simulink model "DataCenterCooling"  (R2026a)
settings: Solver=VariableStepAuto  StopTime=432000  AbsTol=1e-3
PreLoadFcn:
  | load DataCenterCoolingHeatLoad.mat
  | load DataCenterCoolingEnviornment.mat
  | 
  | % Chiller Setpoint
  | T_chiller = 18; % degC
  | 
  | % Pipes
  | server_pipe_D = 0.02; % m
  | server_pipe_L = 12; % m
  | server_pipe_thickness = 0.002; % m
  | server_num_pipes = 800;
  | 
  | % Material properties
  | rho_pipe = 7800; % kg/m^3
  | cp_pipe = 500; % J/(kg*K)
  | 
  | % Total connecting port areas
  | port_area = 0.2; % m^2
  | 
  | % Cooling tower
  | T_reservoir = 23; % degC
  | fan_area = 15; % m^2
  | tower_height = 3; % m
  | tower_area = 15; % m^2
libraries: fl_lib x38, nesl_utility x24, SimscapeFluids_lib x14, simulink_extras x2, slpidlib x2
(part 1 of 2)
CloseFcn:
  | try,close(h1_DataCenterCooling),end
  | clear h1_DataCenterCooling
  | try,close(h2_DataCenterCooling),end
  | clear h2_DataCenterCooling
  | try,close(h3_DataCenterCooling),end
  | clear h3_DataCenterCooling
  | 
  | clear tout simlog_DataCenterCooling
  | clear heat_load environment
  | clear T_chiller server_pipe_D server_pipe_L server_pipe_thickness server_num_pipes
  | clear rho_pipe cp_pipe port_area T_reservoir fan_area tower_height tower_area
Description:
  | Data Center Cooling
settings Model: Creator=The MathWorks, Inc.
settings SolverCC: MaxConsecutiveMinStep=500
settings DataIOCC: ReturnWorkspaceOutputs=on  SignalLogging=on  SaveTime=on  SaveOutput=on
settings DebuggingCC: SymbolicDimsDataTypeCodeGenerationDiagnostic=none
settings SimscapeCC: SimscapeNominalValues="[{\"value\":\"1\",\"unit\":\"A\"},{\"value\":\"1\",\"unit\":\"bar\"},{\"value\":\"1\",\"unit\":\"cm^2\"},{\"value\":\"1\",\"unit\":\"cm^3/s\"},{\"value\":\"1\",\"unit\":\"kJ/kg\"},{\"value\":\"1\",\"unit\":\"kW\"},{\"value\":\"1\",\"unit\":\"l\"},{\"value\":\"1\",\"unit\":\"N\"},{\"value\":\"1\",\"unit\":\"N*m\"},{\"value\":\"1\",\"unit\":\"V\"}]"  SimscapeLogSimulationStatistics=on  SimscapeLogName=simlog_DataCenterCooling  SimscapeLogDataHistory=50000.0

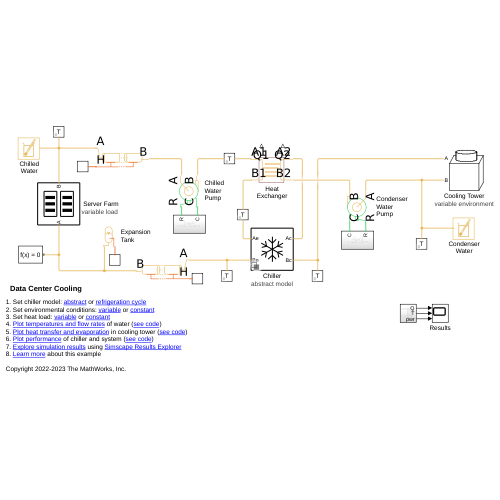
[thumbnail: Simulink's stored preview of the top-level diagram]
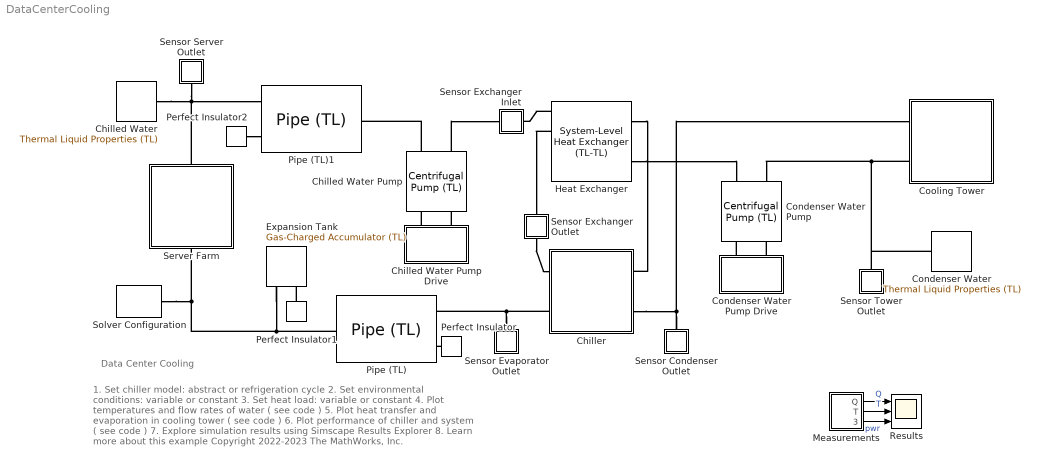
== system DataCenterCooling ==
  note: Data Center Cooling
  note: 1. Set chiller model: abstract or refrigeration cycle
      | 2. Set environmental conditions: variable or constant
      | 3. Set heat load: variable or constant
      | 4. Plot temperatures and flow rates of water ( see code )
      | 5. Plot heat transfer and evaporation in cooling tower ( see code )
      | 6. Plot performance of chiller and system ( see code )
      | 7. Explore simulation results using Simscape Results Explorer
      | 8. Learn more about this example
      |
      | Copyright 2022-2023 The MathWorks, Inc.
  Chilled Water : SimscapeFluids_lib/Thermal Liquid/Utilities/Thermal Liquid Properties (TL)  fluid_list=fluids.thermal_liquid.utilities.enum.thermal_liquid_fluid_list.ethylene_glycol  concentration_param_EG=fluids.thermal_liquid.utilities.enum.thermal_liquid_concentration.volume_fraction  concentration_param_PG=fluids.thermal_liquid.utilities.enum.thermal_liquid_concentration.volume_fraction  c_mass_SW=3.5e-3  c_mass_EG=0.1  c_mass_PG=0.1  c_mass_GL=0.1  c_vol_EG=0.3  c_vol_PG=0.1  beta_const_EG=2.1791 GPa  beta_const_PG=2.1791 GPa  beta_const_GL=2.1791 GPa  p_min_EG=0.01 MPa  p_min_PG=0.01 MPa  p_min_GL=0.01 MPa  p_max_EG=50 MPa  p_max_PG=50 MPa  p_max_GL=50 MPa  T_atm=293.15 K  p_atm=0.101325 MPa  properties_range_check=simscape.enum.assert.action.error  air_fraction=0  R_air=0.287 kJ/(K*kg)  air_dissolution_model=false  p_crit=3 MPa
  Chilled Water Pump : SimscapeFluids_lib/Thermal Liquid/Pumps & Motors/Centrifugal Pump (TL)  pump_parameterization=fluids.thermal_liquid.pumps_motors.enum.CentrifugalPumpParameterization.Nominal  capacity_ref_nominal=9600 lpm  head_ref_nominal=28 m  power_ref_nominal=60 kW  head_ref_max=40 m  capacity_ref_max=15000 lpm  omega_ref_analytic=2400 rpm  flow_rate_1D_TLU=[16.67, 30, 40, 53.33, 66.67, 83.33] lpm  head_1D_TLU=[50, 47.5, 45, 40, 35, 25] m  power_1D_TLU=[.6, .75, .85, .93, .98, .99] kW  omega_ref_1D=3500 rpm  rho_ref_1D=998.21 kg/m^3  omega_threshold_factor=1e-2  flow_rate_2D_TLU=[16.67, 23.33, 30, 40, 53.33, 60] lpm  omega_2D_TLU=[2450, 2800, 3150, 3500] rpm  head_2D_TLU=[25, 32.7, 42.5, 50; 24, 31.7, 41, 49; 22.7, 30.5, 39, 47.5; 20, 28, 36, 45; 15.7, 24, 32, 40; 12.5, 21, 29.5, 37.5] m  power_2D_TLU=[.28, .38, .5, .6; .31, .41, .55, .68; .33, .44, .6, .75; .36, .48, .65, .83; .38, .53, .72, .93; .39, .55, .75, .97] kW  rho_ref_2D=998.21 kg/m^3  diameter_ratio=1  mech_orientation=fluids.thermal_liquid.pumps_motors.enum.CentrifugalPumpMechOrientation.Positive  area=port_area m^2  operation_check=simscape.enum.assert.action.none
  Chilled Water Pump Drive : Subsystem
      settings: PortSchema="{\"entries\":[{\"content\":{\"sides\":[{\"content\":{},\"type\":\"ConnectorPlacement.EquallySpacedRectSide\",\"uuid\":\"edaea338-c02b-45e4-bb82-2d3d355c0ecb\"},{\"content\":{\"side\":\"RIGHT\"},\"type\":\"ConnectorPlacement.EquallySpacedRectSide\",\"uuid\":\"dbf9c5c1-eafd-40d4-aa46-26e8ea9aa192\"},{\"content\":{\"connectorIds\":[\"LConn1\",\"LConn2\"],\"side\":\"TOP\"},\"type\":\"ConnectorPlacement.EquallySpacedRectSide\",\"uuid\":\"608efdba-9ff5-4da4-84d8-d12421fbb1b5\"}]},\"type\":\"ConnectorPlacement.EquallySpacedConnector\",\"uuid\":\"d68ea5d9-0a41-4434-9ea5-6f17886b9eb3\"}],\"packageUris\":[\"http://schema.mathworks.com/mf0/Connector/R2020b\"],\"version\":\"1.0\"}"
  Chiller : Subsystem  Variant=on  VariantControlMode=label  LabelModeActiveChoice=abstract model
      settings: AttributesFormatString=%<LabelModeActiveChoice>
      mask Display:
      | plot([-100 100 100 -100 -100], [-100 -100 100 100 -100])
      | 
      | % Width and height scale factors
      | w = 60;
      | h = 60;
      | 
      | % Coordinates [x; y]
      | trunk = [0 0; -1 1];
      | tip1 = [-0.3 0 0.3; 0.8 0.5 0.8];
      | tip2 = [-0.3 0 0.3; -0.8 -0.5 -0.8];
      | 
      | % Vertical line
      | plot(w*trunk(1,:), h*trunk(2,:))
      | plot(w*tip1(1,:), h*tip1(2,:))
      | plot(w*tip2(1,:), h*tip2(2,:))
      | 
      | % Rotate 60 deg
      | theta = 60;
      | rot = [cosd(theta) -sind(theta); sind(theta) cosd(theta)];
      | trunk_rot = rot*trunk;
      | tip1_rot = rot*tip1;
      | tip2_rot = rot*tip2;
      | plot(w*trunk_rot(1,:), h*trunk_rot(2,:))
      | plot(w*tip1_rot(1,:), h*tip1_rot(2,:))
      | plot(w*tip2_rot(1,:), h*tip2_rot(2,:))
      | 
      | % Rotate 120 deg
      | theta = 120;
      | rot = [cosd(theta) -sind(theta); sind(theta) cosd(theta)];
      | trunk_rot = rot*trunk;
      | tip1_rot = rot*tip1;
      | tip2_rot = rot*tip2;
      | plot(w*trunk_rot(1,:), h*trunk_rot(2,:))
      | plot(w*tip1_rot(1,:), h*tip1_rot(2,:))
      | plot(w*tip2_rot(1,:), h*tip2_rot(2,:))
  Condenser Water : SimscapeFluids_lib/Thermal Liquid/Utilities/Thermal Liquid Properties (TL)  fluid_list=fluids.thermal_liquid.utilities.enum.thermal_liquid_fluid_list.water  concentration_param_EG=fluids.thermal_liquid.utilities.enum.thermal_liquid_concentration.volume_fraction  concentration_param_PG=fluids.thermal_liquid.utilities.enum.thermal_liquid_concentration.volume_fraction  c_mass_SW=3.5e-3  c_mass_EG=0.1  c_mass_PG=0.1  c_mass_GL=0.1  c_vol_EG=0.1  c_vol_PG=0.1  beta_const_EG=2.1791 GPa  beta_const_PG=2.1791 GPa  beta_const_GL=2.1791 GPa  p_min_EG=0.01 MPa  p_min_PG=0.01 MPa  p_min_GL=0.01 MPa  p_max_EG=50 MPa  p_max_PG=50 MPa  p_max_GL=50 MPa  T_atm=293.15 K  p_atm=0.101325 MPa  properties_range_check=simscape.enum.assert.action.error  air_fraction=0  R_air=0.287 kJ/(K*kg)  air_dissolution_model=false  p_crit=3 MPa
  Condenser Water Pump : SimscapeFluids_lib/Thermal Liquid/Pumps & Motors/Centrifugal Pump (TL)  pump_parameterization=fluids.thermal_liquid.pumps_motors.enum.CentrifugalPumpParameterization.Nominal  capacity_ref_nominal=15000 lpm  head_ref_nominal=33 m  power_ref_nominal=100 kW  head_ref_max=48 m  capacity_ref_max=24000 lpm  omega_ref_analytic=2400 rpm  flow_rate_1D_TLU=[16.67, 30, 40, 53.33, 66.67, 83.33] lpm  head_1D_TLU=[50, 47.5, 45, 40, 35, 25] m  power_1D_TLU=[.6, .75, .85, .93, .98, .99] kW  omega_ref_1D=3500 rpm  rho_ref_1D=998.21 kg/m^3  omega_threshold_factor=1e-2  flow_rate_2D_TLU=[16.67, 23.33, 30, 40, 53.33, 60] lpm  omega_2D_TLU=[2450, 2800, 3150, 3500] rpm  head_2D_TLU=[25, 32.7, 42.5, 50; 24, 31.7, 41, 49; 22.7, 30.5, 39, 47.5; 20, 28, 36, 45; 15.7, 24, 32, 40; 12.5, 21, 29.5, 37.5] m  power_2D_TLU=[.28, .38, .5, .6; .31, .41, .55, .68; .33, .44, .6, .75; .36, .48, .65, .83; .38, .53, .72, .93; .39, .55, .75, .97] kW  rho_ref_2D=998.21 kg/m^3  diameter_ratio=1  mech_orientation=fluids.thermal_liquid.pumps_motors.enum.CentrifugalPumpMechOrientation.Positive  area=port_area m^2  operation_check=simscape.enum.assert.action.none
  Condenser Water Pump Drive : Subsystem
      settings: PortSchema="{\"entries\":[{\"content\":{\"sides\":[{\"content\":{},\"type\":\"ConnectorPlacement.EquallySpacedRectSide\",\"uuid\":\"edaea338-c02b-45e4-bb82-2d3d355c0ecb\"},{\"content\":{\"side\":\"RIGHT\"},\"type\":\"ConnectorPlacement.EquallySpacedRectSide\",\"uuid\":\"dbf9c5c1-eafd-40d4-aa46-26e8ea9aa192\"},{\"content\":{\"connectorIds\":[\"LConn1\",\"LConn2\"],\"side\":\"TOP\"},\"type\":\"ConnectorPlacement.EquallySpacedRectSide\",\"uuid\":\"608efdba-9ff5-4da4-84d8-d12421fbb1b5\"}]},\"type\":\"ConnectorPlacement.EquallySpacedConnector\",\"uuid\":\"d68ea5d9-0a41-4434-9ea5-6f17886b9eb3\"}],\"packageUris\":[\"http://schema.mathworks.com/mf0/Connector/R2020b\"],\"version\":\"1.0\"}"
  Cooling Tower : Subsystem  Tag=PublishSubsystem  InitFcn=set_param(gcb, 'AttributesFormatString', get_param([gcb '/Variant Source'], 'LabelModeActiveChoice'))
      settings: AttributesFormatString=variable environment
      mask Display:
      | color('white')
      | plot(100, 100)
      | plot(-100, -100)
      | color('black')
      | 
      | % Number of points on arcs
      | n = 40;
      | 
      | y1 = 80;
      | w1 = 50;
      | h1 = 10;
      | 
      | y2 = 40;
      | y3 = -100;
      | w2 = 70;
      | h2 = 20;
      | 
      | % Cylinder
      | plot([-w1 -w1] + h2/2, [y1 y2])
      | plot([w1 w1] + h2/2, [y1 y2])
      | plot(cos(linspace(0, 2*pi, n))*w1 + h2/2, sin(linspace(0, 2*pi, n))*h1 + y1)
      | plot(cos(linspace(0, pi, n/2))*w1 + h2/2, -sin(linspace(0, pi, n/2))*h1 + y2)
      | 
      | % Box
      | plot([-w2 w2 w2 -w2 -w2], [y2 y2 y3 y3 y2]-h2)
      | plot([-w2+h2 -w1+h2/2], [y2+h2 y2+h2])
      | plot([w1+h2/2 w2+h2 w2+h2], [y2+h2 y2+h2 y3+h2])
      | plot([w2 w2+h2], [y2-h2 y2+h2])
      | plot([w2 w2+h2], [y3-h2 y3+h2])
      | plot([-w2 -w2+h2], [y2-h2 y2+h2])
  Expansion Tank : SimscapeFluids_lib/Thermal Liquid/Tanks & Accumulators/Gas-Charged Accumulator (TL)  capacity=1 m^3  dead_volume=1e-3 m^3  p_precharge_gauge=0.28 MPa  k_sh=1.4  area=port_area m^2  stiff_coeff=1e4 MPa/m^3  damping_coeff=1e4 MPa*s/m^6  liquid_volume_specify=on  liquid_volume_priority=None  liquid_volume=5e-3 m^3  liquid_volume_nominal_specify=off  liquid_volume_nominal_value=1  liquid_volume_nominal_unit=m^3  liquid_mass_specify=off  liquid_mass_priority=None  liquid_mass=5 kg  liquid_mass_nominal_specify=off  liquid_mass_nominal_value=1  liquid_mass_nominal_unit=kg  p_I_specify=on  p_I_priority=High  p_I=0.4 MPa  p_I_nominal_specify=off  p_I_nominal_value=1  p_I_nominal_unit=MPa  T_I_specify=on  T_I_priority=High  T_I=18 degC  T_I_nominal_specify=off  T_I_nominal_value=1  T_I_nominal_unit=K
  Heat Exchanger : SimscapeFluids_lib/Heat Exchangers/Thermal Liquid/System-Level Heat Exchanger (TL-TL)  flow_arrangement=fluids.heat_exchangers.enum.SystemLevelFlowArrangementTLTL.Counter  wall_thermal_mass=false  mass_wall=1 kg  cp_wall=490 J/(K*kg)  nominal_init_wall=true  T_wall_init=293.15 K  area_A1=port_area m^2  area_B1=port_area m^2  area_A2=port_area m^2  area_B2=port_area m^2  operating_condition_TL1=fluids.heat_exchangers.enum.SystemLevelOperatingConditionTLTL.Cooling  mdot_nominal_TL1=160 kg/s  delta_p_nominal_TL1=0.1 MPa  p_in_nominal_TL1=0.6 MPa  T_in_nominal_TL1=28 degC  capacity_spec_TL1=fluids.heat_exchangers.enum.SystemLevelCapacitySpec.HeatTransfer  Q_nominal=3000 kW  T_out_nominal_TL1=323.15 K  volume_TL1=2 m^3  nominal_init_TL1=true  p_init_TL1=0.101325 MPa  T_init_TL1=293.15 K  mdot_nominal_TL2=250 kg/s  delta_p_nominal_TL2=0.2 MPa  p_in_nominal_TL2=0.4 MPa  T_in_nominal_TL2=22 degC  volume_TL2=2 m^3  nominal_init_TL2=true  p_init_TL2=0.101325 MPa  T_init_TL2=293.15 K  a_TL1=0.023  b_TL1=0.8  c_TL1=0.33  a_TL2=0.023  b_TL2=0.8  c_TL2=0.33
  Measurements : Subsystem
  Perfect Insulator : fl_lib/Thermal/Thermal Elements/Perfect Insulator  T_specify=off  T_priority=None  T=293.15 K  T_nominal_specify=off  T_nominal_value=1  T_nominal_unit=K
  Perfect Insulator1 : fl_lib/Thermal/Thermal Elements/Perfect Insulator  T_specify=off  T_priority=None  T=293.15 K  T_nominal_specify=off  T_nominal_value=1  T_nominal_unit=K
  Perfect Insulator2 : fl_lib/Thermal/Thermal Elements/Perfect Insulator  T_specify=off  T_priority=None  T=293.15 K  T_nominal_specify=off  T_nominal_value=1  T_nominal_unit=K
  Pipe (TL) : SimscapeFluids_lib/Thermal Liquid/Pipes & Fittings/Pipe (TL)  dynamic_compressibility=true  inertia=false  num_segments=1  pipe_length=10 m  cross_section_geometry=fluids.thermal_liquid.pipes_fittings.enum.CrossSectionGeometry.Custom  pipe_diameter=0.1 m  pipe_inner_diameter=0.05 m  pipe_outer_diameter=0.1 m  pipe_width=0.1 m  pipe_height=0.1 m  pipe_major_axis=0.1 m  pipe_minor_axis=0.05 m  pipe_side=0.1 m  pipe_angle=30 deg  area=pi*0.05^2/4 * 30 m^2  Dh=0.05 m  elevation_spec=foundation.enum.constant_variable.constant  elevation_gain=0 m  gravity_spec=foundation.enum.constant_variable.constant  g=9.81 m/s^2  pressure_loss_spec=fluids.thermal_liquid.pipes_fittings.enum.PressureLossSpec.Haaland  local_pressure_loss_spec=fluids.thermal_liquid.pipes_fittings.enum.LocalLossSpec.LossCoefficient  length_add=1 m  loss_coefficient=1  roughness_spec=fluids.thermal_liquid.pipes_fittings.enum.RoughnessSpec.Custom  roughness=15e-6 m  Re_friction_TLU=[400, 1000, 1500, 3000, 4000, 6000, 10000, 20000, 40000, 60000, 100000, 100000000]  friction_factor_TLU=[.264, .112, .071, .0417, .0387, .0268, .025, .0232, .0226, .022, .0214, .0214]  Re_lam=2000  Re_tur=4000  shape_factor=64  mdot_nominal=[.1, 1] kg/s  p_diff_nominal=[.001, .01] MPa  mdot_threshold=1e-6 kg/s  wall_spec=fluids.thermal_liquid.pipes_fittings.enum.wall_spec.rigid  vol_expansion_spec=fluids.thermal_liquid.pipes_fittings.enum.VolumeExpansionSpec.Diameter  area_pressure_gain=1e-6 m^2/MPa  static_pressure_TLU=[.1, 1] MPa  area_pressure_gain_TLU=[1e-05, 1.1e-05] m^2  material_behavior_spec=fluids.thermal_liquid.pipes_fittings.enum.PipeMaterialBehavior.Linear  diameter_pressure_gain=1e-6 m/MPa  wall_thickness=0.05 m  elastic_modulus=69 GPa  stress_TLU=[276, 310] MPa  strain_TLU=[.004, .02]  stress_assert_action=simscape.enum.assert.action.none  stress_max=400 MPa  poisson_ratio=0.33  wall_time_constant=0.01 s  thermal_expansion=false  alpha_L_wall=24 um/(deltaK*m)  thermal_expansion_Tref=293.15 K  heat_transfer_spec=fluids.thermal_liquid.pipes_fittings.enum.HeatTransferSpec.Gnielinski  mdot_nominal_heat=[.1, 1] kg/s  T_in_nominal=[293.15, 293.15] K  T_out_nominal=[300, 300] K  p_in_nominal_heat=[.101325, .101325] MPa  T_wall_nominal=[303.15, 303.15] K  a_coeff=0.023  b_Re_power=0.8  c_Pr_power=0.4  Nu_lam=3.66  Re_Colburn_TLU=[100, 150, 1000]  Colburn_factor_TLU=[.019, .013, .002]  Re_Nu_TLU=[100, 150, 1000]  Pr_Nu_TLU=[1, 10]  Nu_TLU=[3.72, 4.21; 3.75, 4.44; 4.21, 7.15]  p0_vec=0.4 MPa  T0_vec=18 degC  mdot0=0.1 kg/s  p_nominal=0.101325 MPa  T_nominal=293.15 K
  Pipe (TL)1 : SimscapeFluids_lib/Thermal Liquid/Pipes & Fittings/Pipe (TL)  dynamic_compressibility=true  inertia=false  num_segments=1  pipe_length=10 m  cross_section_geometry=fluids.thermal_liquid.pipes_fittings.enum.CrossSectionGeometry.Custom  pipe_diameter=0.1 m  pipe_inner_diameter=0.05 m  pipe_outer_diameter=0.1 m  pipe_width=0.1 m  pipe_height=0.1 m  pipe_major_axis=0.1 m  pipe_minor_axis=0.05 m  pipe_side=0.1 m  pipe_angle=30 deg  area=pi*0.05^2/4 * 30 m^2  Dh=0.05 m  elevation_spec=foundation.enum.constant_variable.constant  elevation_gain=0 m  gravity_spec=foundation.enum.constant_variable.constant  g=9.81 m/s^2  pressure_loss_spec=fluids.thermal_liquid.pipes_fittings.enum.PressureLossSpec.Haaland  local_pressure_loss_spec=fluids.thermal_liquid.pipes_fittings.enum.LocalLossSpec.LossCoefficient  length_add=1 m  loss_coefficient=1  roughness_spec=fluids.thermal_liquid.pipes_fittings.enum.RoughnessSpec.Custom  roughness=15e-6 m  Re_friction_TLU=[400, 1000, 1500, 3000, 4000, 6000, 10000, 20000, 40000, 60000, 100000, 100000000]  friction_factor_TLU=[.264, .112, .071, .0417, .0387, .0268, .025, .0232, .0226, .022, .0214, .0214]  Re_lam=2000  Re_tur=4000  shape_factor=64  mdot_nominal=[.1, 1] kg/s  p_diff_nominal=[.001, .01] MPa  mdot_threshold=1e-6 kg/s  wall_spec=fluids.thermal_liquid.pipes_fittings.enum.wall_spec.rigid  vol_expansion_spec=fluids.thermal_liquid.pipes_fittings.enum.VolumeExpansionSpec.Diameter  area_pressure_gain=1e-6 m^2/MPa  static_pressure_TLU=[.1, 1] MPa  area_pressure_gain_TLU=[1e-05, 1.1e-05] m^2  material_behavior_spec=fluids.thermal_liquid.pipes_fittings.enum.PipeMaterialBehavior.Linear  diameter_pressure_gain=1e-6 m/MPa  wall_thickness=0.05 m  elastic_modulus=69 GPa  stress_TLU=[276, 310] MPa  strain_TLU=[.004, .02]  stress_assert_action=simscape.enum.assert.action.none  stress_max=400 MPa  poisson_ratio=0.33  wall_time_constant=0.01 s  thermal_expansion=false  alpha_L_wall=24 um/(deltaK*m)  thermal_expansion_Tref=293.15 K  heat_transfer_spec=fluids.thermal_liquid.pipes_fittings.enum.HeatTransferSpec.Gnielinski  mdot_nominal_heat=[.1, 1] kg/s  T_in_nominal=[293.15, 293.15] K  T_out_nominal=[300, 300] K  p_in_nominal_heat=[.101325, .101325] MPa  T_wall_nominal=[303.15, 303.15] K  a_coeff=0.023  b_Re_power=0.8  c_Pr_power=0.4  Nu_lam=3.66  Re_Colburn_TLU=[100, 150, 1000]  Colburn_factor_TLU=[.019, .013, .002]  Re_Nu_TLU=[100, 150, 1000]  Pr_Nu_TLU=[1, 10]  Nu_TLU=[3.72, 4.21; 3.75, 4.44; 4.21, 7.15]  p0_vec=0.4 MPa  T0_vec=28 degC  mdot0=0.1 kg/s  p_nominal=0.101325 MPa  T_nominal=293.15 K
  Results : Scope  NumInputPorts=3
      settings: Title=Heat Transfer (kW)  ActiveDisplayYMinimum=-2477.8037317681906  ActiveDisplayYMaximum=8330.5842888201569
  Sensor Condenser Outlet : Subsystem
      mask Display: disp('T')
  Sensor Evaporator Outlet : Subsystem
      mask Display: disp('T')
  Sensor Exchanger Inlet : Subsystem
      mask Display: disp('T')
  Sensor Exchanger Outlet : Subsystem
      mask Display: disp('T')
  Sensor Server Outlet : Subsystem
      mask Display: disp('T')
  Sensor Tower Outlet : Subsystem
      mask Display: disp('T')
  Server Farm : Subsystem  Tag=PublishSubsystem  InitFcn=set_param(gcb, 'AttributesFormatString', get_param([gcb '/Variant Source'], 'LabelModeActiveChoice'))
      settings: AttributesFormatString=variable load  PortSchema="{\"entries\":[{\"content\":{\"sides\":[{\"content\":{},\"type\":\"ConnectorPlacement.EquallySpacedRectSide\",\"uuid\":\"edaea338-c02b-45e4-bb82-2d3d355c0ecb\"},{\"content\":{\"side\":\"RIGHT\"},\"type\":\"ConnectorPlacement.EquallySpacedRectSide\",\"uuid\":\"dbf9c5c1-eafd-40d4-aa46-26e8ea9aa192\"},{\"content\":{\"connectorIds\":[\"LConn1\"],\"side\":\"TOP\"},\"type\":\"ConnectorPlacement.EquallySpacedRectSide\",\"uuid\":\"608efdba-9ff5-4da4-84d8-d12421fbb1b5\"},{\"content\":{\"connectorIds\":[\"RConn1\"],\"side\":\"BOTTOM\"},\"type\":\"ConnectorPlacement.EquallySpacedRectSide\",\"uuid\":\"946bb541-0a3a-481c-b51c-306f34404873\"}]},\"type\":\"ConnectorPlacement.EquallySpacedConnector\",\"uuid\":\"d68ea5d9-0a41-4434-9ea5-6f17886b9eb3\"}],\"packageUris\":[\"http://schema.mathworks.com/mf0/Connector/R2020b\"],\"version\":\"1.0\"}"
      mask Display:
      | plot([-100 100 100 -100 -100], [-100 -100 100 100 -100])
      | 
      | dx = 40;
      | 
      | h1 = 120;
      | w1 = 60;
      | 
      | h2 = 10;
      | w2 = 40;
      | 
      | plot([-w1 w1 w1 -w1 -w1]/2 - dx, [h1 h1 -h1 -h1 h1]/2)
      | plot([-w1 w1 w1 -w1 -w1]/2 + dx, [h1 h1 -h1 -h1 h1]/2)
      | 
      | patch([-w2 w2 w2 -w2 -w2]/2 - dx, [h2 h2 -h2 -h2 h2]/2 + h1/4)
      | patch([-w2 w2 w2 -w2 -w2]/2 - dx, [h2 h2 -h2 -h2 h2]/2)
      | patch([-w2 w2 w2 -w2 -w2]/2 - dx, [h2 h2 -h2 -h2 h2]/2 - h1/4)
      | 
      | patch([-w2 w2 w2 -w2 -w2]/2 + dx, [h2 h2 -h2 -h2 h2]/2 + h1/4)
      | patch([-w2 w2 w2 -w2 -w2]/2 + dx, [h2 h2 -h2 -h2 h2]/2)
      | patch([-w2 w2 w2 -w2 -w2]/2 + dx, [h2 h2 -h2 -h2 h2]/2 - h1/4)
  Solver Configuration : nesl_utility/Solver Configuration  PhysicalDomain=network_engine_domain  SubClassName=solver  LeftPortType=input  RightPortType=generic  Tones=[]  Harmonics=[]  SimulateNoise=off  Profile=off  UseLocalSampling=off  EnableSwitchedLinearOptims=on  FrequencyDomain=off  UseCCode=off  RelTol=0.001  AbsTol=0.001  MinStep=1e-09  ToWorkspace=off  RevertToSquareIcSolve=off  NumHomotopyIterations=100  PhasorMode=off  PhasorModeNumHarmonics=1  ConsistencySolver=NEWTON_XTOL_AFTER_FTOL  CanonicalOrdering=UNORDERED  OptimizeIntermediates=UNOPTIMIZED  IndexReductionMethod=None  DoDC=off  ResidualTolerance=1e-09  ConsistencyTolSource=GLOBAL  ConsistencyAbsTol=0.001  ConsistencyRelTol=0.001  ConsistencyTolFactor=0.001  UseLocalSolver=off  LocalSolverChoice=NE_BACKWARD_EULER_ADVANCER  ResolveIndetEquations=on  FunctionEvalNumThread=1  LocalSolverSampleTime=0.001  DoFixedCost=off  MaxNonlinIter=3  MaxModeIter=2  ComputeImpulses=off  ImpulseIterations=2  LinearAlgebra=auto  LinearAlgebraNumThread=0  EquationFormulation=NE_TIME_EF  DelaysMemoryBudget=1024  AutomaticFiltering=on  FilteringTimeConstant=0.001  PartitionStorageMethod=AS_NEEDED  PartitionMemoryBudget=1024  PartitionMethod=ROBUST  MultibodyUseLocalSolver=off  MultibodyLocalSolverChoice=ODE1  MultibodyLocalSolverSampleTime=0.001
  wires:
  Measurements/1(Q) -> Results/1  "Q"
  Measurements/2(T) -> Results/2  "T"
  Measurements/3(pwr) -> Results/3  "pwr"
  connections:
  Server Farm/LConn1 -- Chilled Water/RConn1 -- Sensor Server Outlet/LConn1 -- Pipe (TL)1/LConn1
  Pipe (TL)/RConn1 -- Server Farm/RConn1 -- Solver Configuration/RConn1 -- Expansion Tank/RConn1
  Perfect Insulator/LConn1 -- Pipe (TL)/LConn2
  Perfect Insulator2/LConn1 -- Pipe (TL)1/LConn2
  Perfect Insulator1/LConn1 -- Expansion Tank/RConn2
  Chilled Water Pump/LConn1 -- Pipe (TL)1/RConn1
  Heat Exchanger/LConn1 -- Sensor Exchanger Inlet/RConn1
  Sensor Exchanger Outlet/RConn1 -- Chiller/LConn1
  Chiller/LConn2 -- Sensor Evaporator Outlet/LConn1 -- Pipe (TL)/LConn1
  Chilled Water Pump Drive/LConn1 -- Chilled Water Pump/RConn1
  Chilled Water Pump Drive/LConn2 -- Chilled Water Pump/RConn2
  Heat Exchanger/RConn1 -- Chiller/RConn1
  Heat Exchanger/RConn2 -- Condenser Water Pump/LConn2
  Sensor Condenser Outlet/LConn1 -- Chiller/RConn2 -- Cooling Tower/LConn1
  Cooling Tower/LConn2 -- Condenser Water/RConn1 -- Sensor Tower Outlet/LConn1 -- Condenser Water Pump/LConn1
  Condenser Water Pump Drive/LConn1 -- Condenser Water Pump/RConn2
  Condenser Water Pump Drive/LConn2 -- Condenser Water Pump/RConn1
  Chilled Water Pump/LConn2 -- Sensor Exchanger Inlet/LConn1
  Heat Exchanger/LConn2 -- Sensor Exchanger Outlet/LConn1

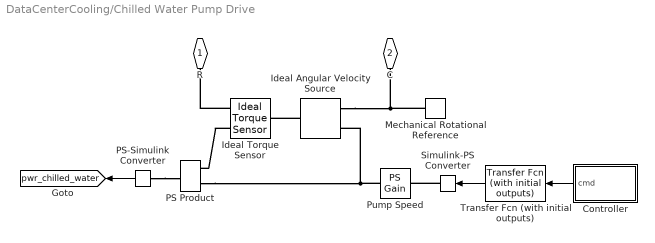
== system DataCenterCooling/Chilled Water Pump Drive ==
  Controller : Subsystem
  Ideal Angular Velocity Source : fl_lib/Mechanical/Mechanical Sources/Ideal Angular Velocity Source
  Ideal Torque Sensor : fl_lib/Mechanical/Mechanical Sensors/Ideal Torque Sensor
  Mechanical Rotational Reference : fl_lib/Mechanical/Rotational Elements/Mechanical Rotational Reference
  PS Product : fl_lib/Physical Signals/Functions/PS Product
  PS-Simulink Converter : nesl_utility/PS-Simulink Converter  PhysicalDomain=network_engine_domain  SubClassName=ps_output  LeftPortType=input  RightPortType=output  PseudoPeriodic=off  Frequencies=[]  VectorFormat=inherit  Unit=kW  AffineConversion=off
  Pump Speed : fl_lib/Physical Signals/Functions/PS Gain  gain=2400 rpm
  Simulink-PS Converter : nesl_utility/Simulink-PS Converter  PhysicalDomain=network_engine_domain  SubClassName=ps_input  LeftPortType=input  RightPortType=output  PseudoPeriodic=off  Frequencies=[]  NoiseDistribution=none  NoiseParameters=[]  Unit=1  AffineConversion=off  FilteringAndDerivatives=provide  SimscapeFilterOrder=1  InputFilterTimeConstant=0.001  UdotUserProvided=0
  Transfer Fcn (with initial outputs) : simulink_extras/Additional Linear/Transfer Fcn (with initial outputs)  N=[1]  D="[2  1]"  Y0=1  U0=0
  R : PMIOPort  Side=Left
  C : PMIOPort  Port=2  Side=Left
  tag scope: pwr_chilled_water=global
  wires:
  Transfer Fcn (with initial outputs)/1 -> Simulink-PS Converter/1
  Controller/1(cmd) -> Transfer Fcn (with initial outputs)/1
  PS-Simulink Converter/1 -> [pwr_chilled_water]
  connections:
  Ideal Angular Velocity Source/RConn2 -- Mechanical Rotational Reference/LConn1 -- C/RConn1
  Pump Speed/RConn1 -- PS Product/LConn2 -- Ideal Angular Velocity Source/RConn1
  Simulink-PS Converter/RConn1 -- Pump Speed/LConn1
  Ideal Angular Velocity Source/LConn1 -- Ideal Torque Sensor/LConn1
  Ideal Torque Sensor/RConn1 -- R/RConn1
  Ideal Torque Sensor/RConn2 -- PS Product/LConn1
  PS-Simulink Converter/LConn1 -- PS Product/RConn1

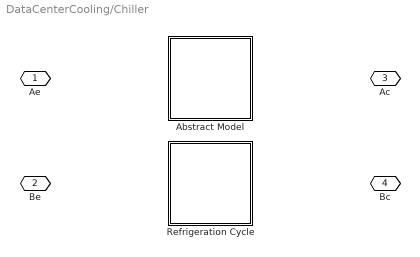
== system DataCenterCooling/Chiller ==
  Abstract Model : Subsystem  Tag=PublishSubsystem  VariantControl=abstract model
  Refrigeration Cycle : Subsystem  Tag=PublishSubsystem  VariantControl=refrigeration cycle
  Ae : PMIOPort  Side=Left
  Be : PMIOPort  Port=2  Side=Left
  Ac : PMIOPort  Port=3  Side=Right
  Bc : PMIOPort  Port=4  Side=Right

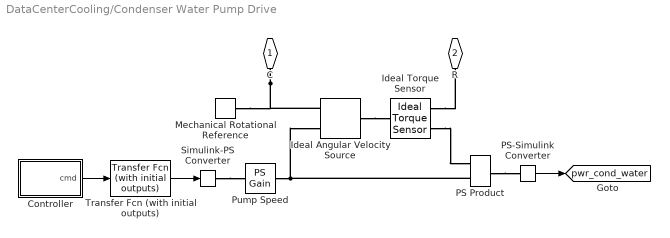
== system DataCenterCooling/Condenser Water Pump Drive ==
  Controller : Subsystem
  Ideal Angular Velocity Source : fl_lib/Mechanical/Mechanical Sources/Ideal Angular Velocity Source
  Ideal Torque Sensor : fl_lib/Mechanical/Mechanical Sensors/Ideal Torque Sensor
  Mechanical Rotational Reference : fl_lib/Mechanical/Rotational Elements/Mechanical Rotational Reference
  PS Product : fl_lib/Physical Signals/Functions/PS Product
  PS-Simulink Converter : nesl_utility/PS-Simulink Converter  PhysicalDomain=network_engine_domain  SubClassName=ps_output  LeftPortType=input  RightPortType=output  PseudoPeriodic=off  Frequencies=[]  VectorFormat=inherit  Unit=kW  AffineConversion=off
  Pump Speed : fl_lib/Physical Signals/Functions/PS Gain  gain=2400 rpm
  Simulink-PS Converter : nesl_utility/Simulink-PS Converter  PhysicalDomain=network_engine_domain  SubClassName=ps_input  LeftPortType=input  RightPortType=output  PseudoPeriodic=off  Frequencies=[]  NoiseDistribution=none  NoiseParameters=[]  Unit=1  AffineConversion=off  FilteringAndDerivatives=provide  SimscapeFilterOrder=1  InputFilterTimeConstant=0.001  UdotUserProvided=0
  Transfer Fcn (with initial outputs) : simulink_extras/Additional Linear/Transfer Fcn (with initial outputs)  N=[1]  D="[2  1]"  Y0=1  U0=0
  C : PMIOPort  Side=Left
  R : PMIOPort  Port=2  Side=Left
  tag scope: pwr_cond_water=global
  wires:
  Transfer Fcn (with initial outputs)/1 -> Simulink-PS Converter/1
  Controller/1(cmd) -> Transfer Fcn (with initial outputs)/1
  PS-Simulink Converter/1 -> [pwr_cond_water]
  connections:
  C/RConn1 -- Ideal Angular Velocity Source/RConn2 -- Mechanical Rotational Reference/LConn1
  Pump Speed/RConn1 -- PS Product/LConn2 -- Ideal Angular Velocity Source/RConn1
  Simulink-PS Converter/RConn1 -- Pump Speed/LConn1
  Ideal Angular Velocity Source/LConn1 -- Ideal Torque Sensor/LConn1
  Ideal Torque Sensor/RConn1 -- R/RConn1
  Ideal Torque Sensor/RConn2 -- PS Product/LConn1
  PS Product/RConn1 -- PS-Simulink Converter/LConn1

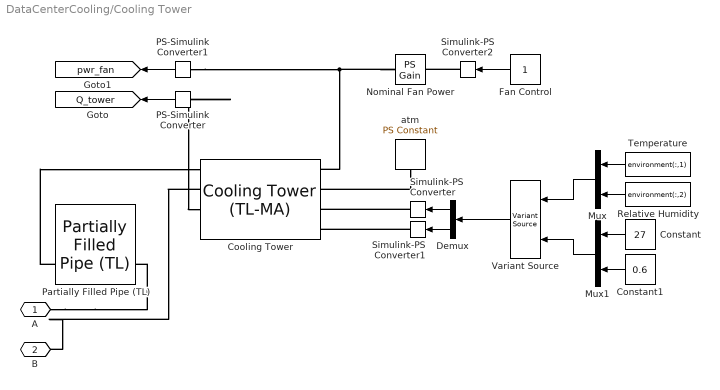
== system DataCenterCooling/Cooling Tower ==
  Constant : Constant  Value=27
  Constant1 : Constant  Value=0.6
  Cooling Tower : SimscapeFluids_lib/Heat Exchangers/Thermal Liquid - Moist Air/Cooling Tower (TL-MA)  flow_arrangement=fluids.heat_exchangers.enum.CoolingTowerFlowArrangement.Counter  capacity_spec_nominal_TL=fluids.heat_exchangers.enum.CoolingTowerCapacitySpecTL.VolumetricFlow  mdot_nominal_TL=42.7 kg/s  q_nominal_TL=15000 lpm  Q_tower_nominal=1000 kW  Q_evap_nominal=800 kW  T_in_nominal_TL=28 degC  T_out_nominal_TL=22 degC  basin_model_TL=true  basin_area_TL=tower_area m^2  area_A1=port_area m^2  area_B1=port_area m^2  drift_rate_TL=0  auto_replenish_TL=true  T_makeup_TL=T_reservoir degC  nominal_init_TL=true  T_init_TL=29.44 degC  level_init_TL=0.5 m  g_TL=9.81 m/s^2  operating_conditions_MA=fluids.heat_exchangers.enum.CoolingTowerOperatingConditionsMA.InputSignals  flow_rate_spec_MA=fluids.heat_exchangers.enum.CoolingTowerFlowRateSpecMA.FanPower  output_power_MA=false  power_nominal_MA=45 kW  humidity_spec_MA=foundation.enum.HumiditySpec.RelativeHumidity  input_error_spec_MA=foundation.enum.input_range_error.warn  full_nominal_condition_MA=true  flow_rate_spec_nominal_MA=foundation.enum.mass_volumetric_flow.volumetric  mdot_nominal_MA=36 kg/s  q_nominal_MA=218 m^3/s  delta_p_nominal_MA=250 Pa  p_in_nominal_MA=0.101325 MPa  T_in_nominal_MA=27 degC  humidity_spec_nominal_MA=foundation.enum.HumiditySpec.RelativeHumidity  RH_in_nominal_MA=0.6  x_w_in_nominal_MA=0.0167  y_w_in_nominal_MA=0.0266  HR_in_nominal_MA=0.017  Tw_in_nominal_MA=25.56 degC  trace_gas_spec_nominal_MA=foundation.enum.trace_gas_spec.mass_fraction  x_g_in_nominal_MA=6e-4  y_g_in_nominal_MA=4e-4  volume_MA=24 m^3  area_A2=4 m^2  area_B2=4 m^2  nominal_init_MA=true  p_init_MA=0.101325 MPa  T_init_MA=34.28 degC  humidity_spec_init_MA=foundation.enum.HumiditySpec.WetBulbTemperature  RH_init_MA=0.5  x_w_init_MA=0.0167  y_w_init_MA=0.0266  HR_init_MA=0.017  Tw_init_MA=25.56 degC  trace_gas_spec_init_MA=foundation.enum.trace_gas_spec.mass_fraction  x_g_init_MA=6e-4  y_g_init_MA=4e-4  r_d_init_MA=0  RH_ws_MA=1  time_constant_cond_MA=1e-3 s  time_constant_evap_MA=1e-3 s  fraction_entrained_MA=1
  Demux : Demux  Outputs=2
  Fan Control : Constant
  Mux : Mux  Inputs=2
  Mux1 : Mux  Inputs=2
  Nominal Fan Power : fl_lib/Physical Signals/Functions/PS Gain  gain=45 kW
  PS-Simulink Converter : nesl_utility/PS-Simulink Converter  PhysicalDomain=network_engine_domain  SubClassName=ps_output  LeftPortType=input  RightPortType=output  PseudoPeriodic=off  Frequencies=[]  VectorFormat=inherit  Unit=kW  AffineConversion=off
  PS-Simulink Converter1 : nesl_utility/PS-Simulink Converter  PhysicalDomain=network_engine_domain  SubClassName=ps_output  LeftPortType=input  RightPortType=output  PseudoPeriodic=off  Frequencies=[]  VectorFormat=inherit  Unit=kW  AffineConversion=off
  Partially Filled Pipe (TL) : SimscapeFluids_lib/Thermal Liquid/Pipes & Fittings/Partially Filled Pipe (TL)  length=tower_height m  area=port_area m^2  Dh=sqrt(4*port_area/pi) m  elevation_drop=tower_height m  level_init=tower_height m  level_check=simscape.enum.assert.action.error  g=9.81 m/s^2  length_add=1 m  roughness=15e-6 m  Re_lam=2000  Re_tur=4000  shape_factor=64  T0=28 degC
  Relative Humidity : FromWorkspace  VariableName=environment(:,2)  OutDataTypeStr=double  OutputAfterFinalValue=Holding final value
  Simulink-PS Converter : nesl_utility/Simulink-PS Converter  PhysicalDomain=network_engine_domain  SubClassName=ps_input  LeftPortType=input  RightPortType=output  PseudoPeriodic=off  Frequencies=[]  NoiseDistribution=none  NoiseParameters=[]  Unit=degC  AffineConversion=on  FilteringAndDerivatives=provide  SimscapeFilterOrder=1  InputFilterTimeConstant=0.001  UdotUserProvided=0
  Simulink-PS Converter1 : nesl_utility/Simulink-PS Converter  PhysicalDomain=network_engine_domain  SubClassName=ps_input  LeftPortType=input  RightPortType=output  PseudoPeriodic=off  Frequencies=[]  NoiseDistribution=none  NoiseParameters=[]  Unit=1  AffineConversion=off  FilteringAndDerivatives=provide  SimscapeFilterOrder=1  InputFilterTimeConstant=0.001  UdotUserProvided=0
  Simulink-PS Converter2 : nesl_utility/Simulink-PS Converter  PhysicalDomain=network_engine_domain  SubClassName=ps_input  LeftPortType=input  RightPortType=output  PseudoPeriodic=off  Frequencies=[]  NoiseDistribution=none  NoiseParameters=[]  Unit=1  AffineConversion=off  FilteringAndDerivatives=provide  SimscapeFilterOrder=1  InputFilterTimeConstant=0.001  UdotUserProvided=0
  Temperature : FromWorkspace  VariableName=environment(:,1)  OutputAfterFinalValue=Holding final value
  Variant Source : VariantSource  VariantControlMode=label  LabelModeActiveChoice=variable environment  VariantControls={variable environment, constant environment}
      settings: AttributesFormatString=%<LabelModeActiveChoice>
  atm : fl_lib/Physical Signals/Sources/PS Constant  constant=1 atm
  A : PMIOPort  Side=Left
  B : PMIOPort  Port=2  Side=Left
  tag scope: Q_tower=global, pwr_fan=global
  wires:
  Temperature/1 -> Mux/1
  Relative Humidity/1 -> Mux/2
  Constant/1 -> Mux1/1
  Constant1/1 -> Mux1/2
  Mux/1 -> Variant Source/1
  Mux1/1 -> Variant Source/2
  Demux/1 -> Simulink-PS Converter/1
  Demux/2 -> Simulink-PS Converter1/1
  Variant Source/1 -> Demux/1
  Fan Control/1 -> Simulink-PS Converter2/1
  PS-Simulink Converter/1 -> [Q_tower]
  PS-Simulink Converter1/1 -> [pwr_fan]
  connections:
  Simulink-PS Converter/RConn1 -- Cooling Tower/RConn3
  Simulink-PS Converter1/RConn1 -- Cooling Tower/RConn4
  Partially Filled Pipe (TL)/LConn2 -- Cooling Tower/LConn1
  Nominal Fan Power/RConn1 -- Cooling Tower/RConn1 -- PS-Simulink Converter1/LConn1
  Simulink-PS Converter2/RConn1 -- Nominal Fan Power/LConn1
  atm/RConn1 -- Cooling Tower/RConn2
  PS-Simulink Converter/LConn1 -- Cooling Tower/LConn3
  Cooling Tower/LConn2 -- B/RConn1
  A/RConn1 -- Partially Filled Pipe (TL)/RConn2

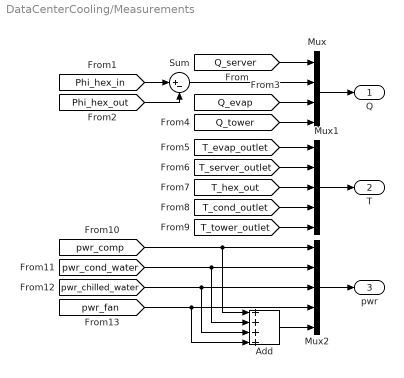
== system DataCenterCooling/Measurements ==
  Add : Sum  Inputs=++++
  Mux : Mux
  Mux1 : Mux  Inputs=5
  Mux2 : Mux  Inputs=5
  Sum : Sum  Inputs=|+-
  Q : Outport
  T : Outport  Port=2
  pwr : Outport  Port=3
  wires:
  [Phi_hex_in] -> Sum/1
  [Phi_hex_out] -> Sum/2
  [Q_server] -> Mux/1
  Sum/1 -> Mux/2
  [Q_evap] -> Mux/3
  [Q_tower] -> Mux/4
  Mux/1 -> Q/1
  [T_evap_outlet] -> Mux1/1
  [T_server_outlet] -> Mux1/2
  [T_hex_out] -> Mux1/3
  [T_cond_outlet] -> Mux1/4
  [T_tower_outlet] -> Mux1/5
  Mux1/1 -> T/1
  [pwr_comp] -> Add/1, Mux2/1
  [pwr_cond_water] -> Add/2, Mux2/2
  [pwr_chilled_water] -> Add/3, Mux2/3
  [pwr_fan] -> Add/4, Mux2/4
  Add/1 -> Mux2/5
  Mux2/1 -> pwr/1

== system DataCenterCooling/Sensor Condenser Outlet ==
  PS-Simulink Converter : nesl_utility/PS-Simulink Converter  PhysicalDomain=network_engine_domain  SubClassName=ps_output  LeftPortType=input  RightPortType=output  PseudoPeriodic=off  Frequencies=[]  VectorFormat=inherit  Unit=degC  AffineConversion=on
  Pressure & Temperature Sensor (TL) : fl_lib/Thermal Liquid/Sensors/Pressure & Temperature Sensor (TL)  reference=foundation.enum.MeasurementReference.absolute  pressure=true  pressure_spec=foundation.enum.PressureMeasementSpec.Absolute  temperature=true
  A : PMIOPort  Side=Left
  tag scope: T_cond_outlet=global
  wires:
  PS-Simulink Converter/1 -> [T_cond_outlet]
  connections:
  Pressure & Temperature Sensor (TL)/RConn2 -- PS-Simulink Converter/LConn1
  Pressure & Temperature Sensor (TL)/LConn1 -- A/RConn1

== system DataCenterCooling/Sensor Evaporator Outlet ==
  PS-Simulink Converter : nesl_utility/PS-Simulink Converter  PhysicalDomain=network_engine_domain  SubClassName=ps_output  LeftPortType=input  RightPortType=output  PseudoPeriodic=off  Frequencies=[]  VectorFormat=inherit  Unit=degC  AffineConversion=on
  Pressure & Temperature Sensor (TL) : fl_lib/Thermal Liquid/Sensors/Pressure & Temperature Sensor (TL)  reference=foundation.enum.MeasurementReference.absolute  pressure=true  pressure_spec=foundation.enum.PressureMeasementSpec.Absolute  temperature=true
  A : PMIOPort  Side=Left
  tag scope: T_evap_outlet=global
  wires:
  PS-Simulink Converter/1 -> [T_evap_outlet]
  connections:
  PS-Simulink Converter/LConn1 -- Pressure & Temperature Sensor (TL)/RConn2
  Pressure & Temperature Sensor (TL)/LConn1 -- A/RConn1

== system DataCenterCooling/Sensor Exchanger Inlet ==
  Flow Rate Sensor (TL) : fl_lib/Thermal Liquid/Sensors/Flow Rate Sensor (TL)  mass_flow_measure=true  volumetric_flow_measure=false  energy_flow_measure=true
  PS-Simulink Converter : nesl_utility/PS-Simulink Converter  PhysicalDomain=network_engine_domain  SubClassName=ps_output  LeftPortType=input  RightPortType=output  PseudoPeriodic=off  Frequencies=[]  VectorFormat=inherit  Unit=kW  AffineConversion=off
  A : PMIOPort  Side=Left
  B : PMIOPort  Port=2  Side=Right
  tag scope: Phi_hex_in=global
  wires:
  PS-Simulink Converter/1 -> [Phi_hex_in]
  connections:
  Flow Rate Sensor (TL)/RConn1 -- B/RConn1
  Flow Rate Sensor (TL)/LConn1 -- A/RConn1
  Flow Rate Sensor (TL)/RConn3 -- PS-Simulink Converter/LConn1

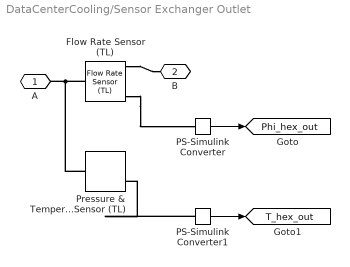
== system DataCenterCooling/Sensor Exchanger Outlet ==
  Flow Rate Sensor (TL) : fl_lib/Thermal Liquid/Sensors/Flow Rate Sensor (TL)  mass_flow_measure=true  volumetric_flow_measure=false  energy_flow_measure=true
  PS-Simulink Converter : nesl_utility/PS-Simulink Converter  PhysicalDomain=network_engine_domain  SubClassName=ps_output  LeftPortType=input  RightPortType=output  PseudoPeriodic=off  Frequencies=[]  VectorFormat=inherit  Unit=kW  AffineConversion=off
  PS-Simulink Converter1 : nesl_utility/PS-Simulink Converter  PhysicalDomain=network_engine_domain  SubClassName=ps_output  LeftPortType=input  RightPortType=output  PseudoPeriodic=off  Frequencies=[]  VectorFormat=inherit  Unit=degC  AffineConversion=on
  Pressure & Temperature Sensor (TL) : fl_lib/Thermal Liquid/Sensors/Pressure & Temperature Sensor (TL)  reference=foundation.enum.MeasurementReference.absolute  pressure=true  pressure_spec=foundation.enum.PressureMeasementSpec.Absolute  temperature=true
  A : PMIOPort  Side=Left
  B : PMIOPort  Port=2  Side=Right
  tag scope: Phi_hex_out=global, T_hex_out=global
  wires:
  PS-Simulink Converter/1 -> [Phi_hex_out]
  PS-Simulink Converter1/1 -> [T_hex_out]
  connections:
  Flow Rate Sensor (TL)/RConn3 -- PS-Simulink Converter/LConn1
  Flow Rate Sensor (TL)/RConn1 -- B/RConn1
  Pressure & Temperature Sensor (TL)/LConn1 -- Flow Rate Sensor (TL)/LConn1 -- A/RConn1
  PS-Simulink Converter1/LConn1 -- Pressure & Temperature Sensor (TL)/RConn2

== system DataCenterCooling/Sensor Server Outlet ==
  PS-Simulink Converter : nesl_utility/PS-Simulink Converter  PhysicalDomain=network_engine_domain  SubClassName=ps_output  LeftPortType=input  RightPortType=output  PseudoPeriodic=off  Frequencies=[]  VectorFormat=inherit  Unit=degC  AffineConversion=on
  Pressure & Temperature Sensor (TL) : fl_lib/Thermal Liquid/Sensors/Pressure & Temperature Sensor (TL)  reference=foundation.enum.MeasurementReference.absolute  pressure=true  pressure_spec=foundation.enum.PressureMeasementSpec.Absolute  temperature=true
  A : PMIOPort  Side=Left
  tag scope: T_server_outlet=global
  wires:
  PS-Simulink Converter/1 -> [T_server_outlet]
  connections:
  Pressure & Temperature Sensor (TL)/LConn1 -- A/RConn1
  Pressure & Temperature Sensor (TL)/RConn2 -- PS-Simulink Converter/LConn1

== system DataCenterCooling/Sensor Tower Outlet ==
  PS-Simulink Converter : nesl_utility/PS-Simulink Converter  PhysicalDomain=network_engine_domain  SubClassName=ps_output  LeftPortType=input  RightPortType=output  PseudoPeriodic=off  Frequencies=[]  VectorFormat=inherit  Unit=degC  AffineConversion=on
  Pressure & Temperature Sensor (TL) : fl_lib/Thermal Liquid/Sensors/Pressure & Temperature Sensor (TL)  reference=foundation.enum.MeasurementReference.absolute  pressure=true  pressure_spec=foundation.enum.PressureMeasementSpec.Absolute  temperature=true
  A : PMIOPort  Side=Left
  tag scope: T_tower_outlet=global
  wires:
  PS-Simulink Converter/1 -> [T_tower_outlet]
  connections:
  PS-Simulink Converter/LConn1 -- Pressure & Temperature Sensor (TL)/RConn2
  Pressure & Temperature Sensor (TL)/LConn1 -- A/RConn1

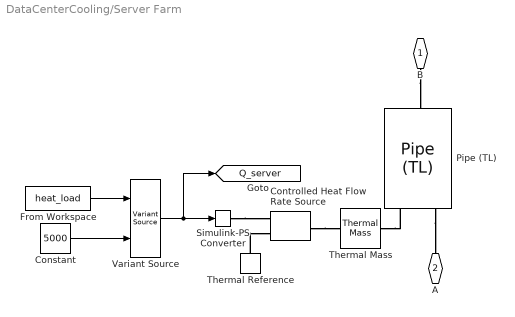
== system DataCenterCooling/Server Farm ==
  Constant : Constant  Value=5000
  Controlled Heat Flow Rate Source : fl_lib/Thermal/Thermal Sources/Controlled Heat Flow Rate Source
  From Workspace : FromWorkspace  VariableName=heat_load  OutputAfterFinalValue=Holding final value
  Pipe (TL) : SimscapeFluids_lib/Thermal Liquid/Pipes & Fittings/Pipe (TL)  dynamic_compressibility=true  inertia=false  num_segments=1  pipe_length=server_pipe_L m  cross_section_geometry=fluids.thermal_liquid.pipes_fittings.enum.CrossSectionGeometry.Custom  pipe_diameter=0.1 m  pipe_inner_diameter=0.05 m  pipe_outer_diameter=0.1 m  pipe_width=0.1 m  pipe_height=0.1 m  pipe_major_axis=0.1 m  pipe_minor_axis=0.05 m  pipe_side=0.1 m  pipe_angle=30 deg  area=pi*server_pipe_D^2/4 * server_num_pipes m^2  Dh=server_pipe_D m  elevation_spec=foundation.enum.constant_variable.constant  elevation_gain=0 m  gravity_spec=foundation.enum.constant_variable.constant  g=9.81 m/s^2  pressure_loss_spec=fluids.thermal_liquid.pipes_fittings.enum.PressureLossSpec.Haaland  local_pressure_loss_spec=fluids.thermal_liquid.pipes_fittings.enum.LocalLossSpec.LossCoefficient  length_add=1 m  loss_coefficient=1  roughness_spec=fluids.thermal_liquid.pipes_fittings.enum.RoughnessSpec.Custom  roughness=15e-6 m  Re_friction_TLU=[400, 1000, 1500, 3000, 4000, 6000, 10000, 20000, 40000, 60000, 100000, 100000000]  friction_factor_TLU=[.264, .112, .071, .0417, .0387, .0268, .025, .0232, .0226, .022, .0214, .0214]  Re_lam=2000  Re_tur=4000  shape_factor=64  mdot_nominal=[.1, 1] kg/s  p_diff_nominal=[.001, .01] MPa  mdot_threshold=1e-6 kg/s  wall_spec=fluids.thermal_liquid.pipes_fittings.enum.wall_spec.rigid  vol_expansion_spec=fluids.thermal_liquid.pipes_fittings.enum.VolumeExpansionSpec.Diameter  area_pressure_gain=1e-6 m^2/MPa  static_pressure_TLU=[.1, 1] MPa  area_pressure_gain_TLU=[1e-05, 1.1e-05] m^2  material_behavior_spec=fluids.thermal_liquid.pipes_fittings.enum.PipeMaterialBehavior.Linear  diameter_pressure_gain=1e-6 m/MPa  wall_thickness=0.05 m  elastic_modulus=69 GPa  stress_TLU=[276, 310] MPa  strain_TLU=[.004, .02]  stress_assert_action=simscape.enum.assert.action.none  stress_max=400 MPa  poisson_ratio=0.33  wall_time_constant=0.01 s  thermal_expansion=false  alpha_L_wall=24 um/(deltaK*m)  thermal_expansion_Tref=293.15 K  heat_transfer_spec=fluids.thermal_liquid.pipes_fittings.enum.HeatTransferSpec.Gnielinski  mdot_nominal_heat=[.1, 1] kg/s  T_in_nominal=[293.15, 293.15] K  T_out_nominal=[300, 300] K  p_in_nominal_heat=[.101325, .101325] MPa  T_wall_nominal=[303.15, 303.15] K  a_coeff=0.023  b_Re_power=0.8  c_Pr_power=0.4  Nu_lam=3.66  Re_Colburn_TLU=[100, 150, 1000]  Colburn_factor_TLU=[.019, .013, .002]  Re_Nu_TLU=[100, 150, 1000]  Pr_Nu_TLU=[1, 10]  Nu_TLU=[3.72, 4.21; 3.75, 4.44; 4.21, 7.15]  p0_vec=0.4 MPa  T0_vec=28 degC  mdot0=0.1 kg/s  p_nominal=0.101325 MPa  T_nominal=293.15 K
  Simulink-PS Converter : nesl_utility/Simulink-PS Converter  PhysicalDomain=network_engine_domain  SubClassName=ps_input  LeftPortType=input  RightPortType=output  PseudoPeriodic=off  Frequencies=[]  NoiseDistribution=none  NoiseParameters=[]  Unit=kW  AffineConversion=off  FilteringAndDerivatives=provide  SimscapeFilterOrder=1  InputFilterTimeConstant=0.001  UdotUserProvided=0
  Thermal Mass : fl_lib/Thermal/Thermal Elements/Thermal Mass  mass_type=foundation.enum.constant_variable.constant  mass=pi*server_pipe_D*server_pipe_L*server_pipe_thickness * server_num_pipes * rho_pipe kg  sp_heat=cp_pipe J/(K*kg)  mass_min=1e-6 kg  num_ports=foundation.enum.numPorts2.two  m_specify=off  m_priority=High  m=1 kg  m_nominal_specify=off  m_nominal_value=1  m_nominal_unit=kg  T_specify=on  T_priority=High  T=28 degC  T_nominal_specify=off  T_nominal_value=1  T_nominal_unit=K  Q_specify=off  Q_priority=None  Q=0 W  Q_nominal_specify=off  Q_nominal_value=1  Q_nominal_unit=W
  Thermal Reference : fl_lib/Thermal/Thermal Elements/Thermal Reference
  Variant Source : VariantSource  VariantControlMode=label  LabelModeActiveChoice=variable load  VariantControls={variable load, constant load}
      settings: AttributesFormatString=%<LabelModeActiveChoice>
  B : PMIOPort  Side=Left
  A : PMIOPort  Port=2  Side=Right
  tag scope: Q_server=global
  wires:
  Variant Source/1 -> [Q_server], Simulink-PS Converter/1
  From Workspace/1 -> Variant Source/1
  Constant/1 -> Variant Source/2
  connections:
  Pipe (TL)/LConn1 -- A/RConn1
  B/RConn1 -- Pipe (TL)/RConn1
  Thermal Mass/RConn1 -- Pipe (TL)/LConn2
  Controlled Heat Flow Rate Source/LConn1 -- Thermal Mass/LConn1
  Thermal Reference/LConn1 -- Controlled Heat Flow Rate Source/RConn2
  Simulink-PS Converter/RConn1 -- Controlled Heat Flow Rate Source/RConn1

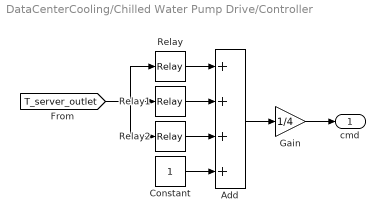
== system DataCenterCooling/Chilled Water Pump Drive/Controller ==
  Add : Sum  Inputs=++++
  Constant : Constant
  Gain : Gain  Gain=1/4
  Relay : Relay  OnSwitchValue=28  OffSwitchValue=24  ZeroCross=off
  Relay1 : Relay  OnSwitchValue=24  OffSwitchValue=20  ZeroCross=off
  Relay2 : Relay  OnSwitchValue=20  OffSwitchValue=16  ZeroCross=off
  cmd : Outport
  wires:
  Relay/1 -> Add/1
  Relay1/1 -> Add/2
  Relay2/1 -> Add/3
  Constant/1 -> Add/4
  [T_server_outlet] -> Relay1/1, Relay/1, Relay2/1
  Add/1 -> Gain/1
  Gain/1 -> cmd/1

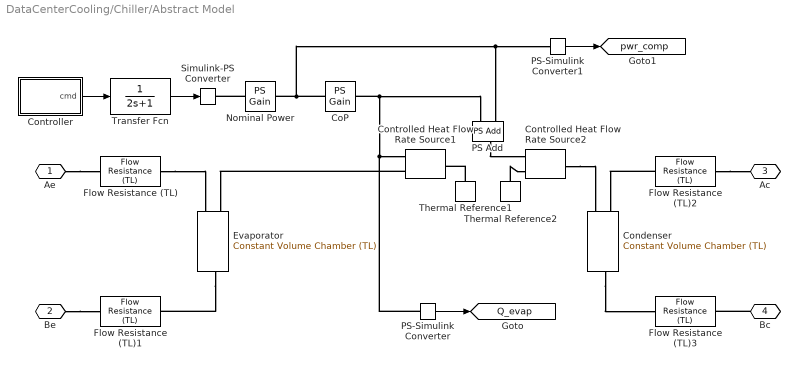
== system DataCenterCooling/Chiller/Abstract Model ==
  CoP : fl_lib/Physical Signals/Functions/PS Gain  gain=13
  Condenser : fl_lib/Thermal Liquid/Elements/Constant Volume Chamber (TL)  volume=0.75 m^3  num_ports=foundation.enum.num_ports.two  area_A=port_area m^2  area_B=port_area m^2  area_C=0.01 m^2  area_D=0.01 m^2  p_I_specify=on  p_I_priority=High  p_I=0.101325 + 0.01 MPa  p_I_nominal_specify=off  p_I_nominal_value=1  p_I_nominal_unit=MPa  T_I_specify=on  T_I_priority=High  T_I=28 degC  T_I_nominal_specify=off  T_I_nominal_value=1  T_I_nominal_unit=K  u_I_specify=off  u_I_priority=None  u_I=83.906 kJ/kg  u_I_nominal_specify=off  u_I_nominal_value=1  u_I_nominal_unit=kJ/kg  rho_I_specify=off  rho_I_priority=None  rho_I=998.21 kg/m^3  rho_I_nominal_specify=off  rho_I_nominal_value=1  rho_I_nominal_unit=kg/m^3
  Controlled Heat Flow Rate Source1 : fl_lib/Thermal/Thermal Sources/Controlled Heat Flow Rate Source
  Controlled Heat Flow Rate Source2 : fl_lib/Thermal/Thermal Sources/Controlled Heat Flow Rate Source
  Controller : Subsystem
  Evaporator : fl_lib/Thermal Liquid/Elements/Constant Volume Chamber (TL)  volume=0.75 m^3  num_ports=foundation.enum.num_ports.two  area_A=port_area m^2  area_B=port_area m^2  area_C=0.01 m^2  area_D=0.01 m^2  p_I_specify=on  p_I_priority=High  p_I=0.4 MPa  p_I_nominal_specify=off  p_I_nominal_value=1  p_I_nominal_unit=MPa  T_I_specify=on  T_I_priority=High  T_I=18 degC  T_I_nominal_specify=off  T_I_nominal_value=1  T_I_nominal_unit=K  u_I_specify=off  u_I_priority=None  u_I=83.906 kJ/kg  u_I_nominal_specify=off  u_I_nominal_value=1  u_I_nominal_unit=kJ/kg  rho_I_specify=off  rho_I_priority=None  rho_I=998.21 kg/m^3  rho_I_nominal_specify=off  rho_I_nominal_value=1  rho_I_nominal_unit=kg/m^3
  Flow Resistance (TL) : fl_lib/Thermal Liquid/Elements/Flow Resistance (TL)  delta_p_nominal=0.1 / 2 MPa  mdot_nominal=185 kg/s  area=port_area m^2  laminar_fraction=1e-3
  Flow Resistance (TL)1 : fl_lib/Thermal Liquid/Elements/Flow Resistance (TL)  delta_p_nominal=0.1 / 2 MPa  mdot_nominal=185 kg/s  area=port_area m^2  laminar_fraction=1e-3
  Flow Resistance (TL)2 : fl_lib/Thermal Liquid/Elements/Flow Resistance (TL)  delta_p_nominal=0.1 / 2 MPa  mdot_nominal=250 kg/s  area=port_area m^2  laminar_fraction=1e-3
  Flow Resistance (TL)3 : fl_lib/Thermal Liquid/Elements/Flow Resistance (TL)  delta_p_nominal=0.1 / 2 MPa  mdot_nominal=250 kg/s  area=port_area m^2  laminar_fraction=1e-3
  Nominal Power : fl_lib/Physical Signals/Functions/PS Gain  gain=270 kW
  PS Add : fl_lib/Physical Signals/Functions/PS Add
  PS-Simulink Converter : nesl_utility/PS-Simulink Converter  PhysicalDomain=network_engine_domain  SubClassName=ps_output  LeftPortType=input  RightPortType=output  PseudoPeriodic=off  Frequencies=[]  VectorFormat=inherit  Unit=kW  AffineConversion=off
  PS-Simulink Converter1 : nesl_utility/PS-Simulink Converter  PhysicalDomain=network_engine_domain  SubClassName=ps_output  LeftPortType=input  RightPortType=output  PseudoPeriodic=off  Frequencies=[]  VectorFormat=inherit  Unit=kW  AffineConversion=off
  Simulink-PS Converter : nesl_utility/Simulink-PS Converter  PhysicalDomain=network_engine_domain  SubClassName=ps_input  LeftPortType=input  RightPortType=output  PseudoPeriodic=off  Frequencies=[]  NoiseDistribution=none  NoiseParameters=[]  Unit=1  AffineConversion=off  FilteringAndDerivatives=provide  SimscapeFilterOrder=1  InputFilterTimeConstant=0.001  UdotUserProvided=0
  Thermal Reference1 : fl_lib/Thermal/Thermal Elements/Thermal Reference
  Thermal Reference2 : fl_lib/Thermal/Thermal Elements/Thermal Reference
  Transfer Fcn : TransferFcn  Denominator=[2 1]
  Ae : PMIOPort  Side=Left
  Be : PMIOPort  Port=2  Side=Left
  Ac : PMIOPort  Port=3  Side=Right
  Bc : PMIOPort  Port=4  Side=Right
  tag scope: Q_evap=global, pwr_comp=global
  wires:
  PS-Simulink Converter1/1 -> [pwr_comp]
  PS-Simulink Converter/1 -> [Q_evap]
  Controller/1(cmd) -> Transfer Fcn/1
  Transfer Fcn/1 -> Simulink-PS Converter/1
  connections:
  Be/RConn1 -- Flow Resistance (TL)1/RConn1
  Thermal Reference2/LConn1 -- Controlled Heat Flow Rate Source2/RConn2
  Ae/RConn1 -- Flow Resistance (TL)/LConn1
  Flow Resistance (TL)2/LConn1 -- Ac/RConn1
  Bc/RConn1 -- Flow Resistance (TL)3/RConn1
  Thermal Reference1/LConn1 -- Controlled Heat Flow Rate Source1/LConn1
  Nominal Power/LConn1 -- Simulink-PS Converter/RConn1
  CoP/LConn1 -- PS Add/LConn1 -- PS-Simulink Converter1/LConn1 -- Nominal Power/RConn1
  PS Add/LConn2 -- CoP/RConn1 -- PS-Simulink Converter/LConn1 -- Controlled Heat Flow Rate Source1/RConn1
  PS Add/RConn1 -- Controlled Heat Flow Rate Source2/RConn1
  Condenser/RConn1 -- Flow Resistance (TL)3/LConn1
  Evaporator/RConn1 -- Flow Resistance (TL)1/LConn1
  Flow Resistance (TL)/RConn1 -- Evaporator/LConn1
  Flow Resistance (TL)2/RConn1 -- Condenser/LConn1
  Controlled Heat Flow Rate Source1/RConn2 -- Evaporator/LConn2
  Controlled Heat Flow Rate Source2/LConn1 -- Condenser/LConn2
